simulink model "HapticPaddle"  (R2025a)
settings: Solver=FixedStepAuto  StartTime=0.0  StopTime=10  FixedStep=0.0001  RelTol=1e-3  EnableMultiTasking=on
values from neighbouring files (symbols this model uses):
  B_eq = B_p + R^2*B_m    (= 0.00017775)    [main.m]
  g = 9.81    [main.m]
  J_eq = (J_p + R^2*(J_rotor + J_m))    (= 0.000485304)    [main.m]
  l = 0.0251    [main.m]
  m_p = 0.048    [main.m]
  phi_target = 10.00    (= 10)    [main.m]
  R = r_p1 / r_m    (= 15)    [main.m]
  r_p2 = 0.081    [main.m]
  Tau_f_dry = 0.00156    [main.m]
libraries: simulink_extras x3
settings Model: Creator=jemetzge  LastModifiedBy=tk
settings SolverCC: AlgebraicLoopSolver=TrustRegion
settings DataIOCC: LimitDataPoints=on  SaveFormat=Array  SignalLoggingSaveFormat=ModelDataLogs  ReturnWorkspaceOutputs=off
settings OptimizationCC: ExpressionDepthLimit=2147483647.0  LifeSpan=inf
settings DebuggingCC: UnderspecifiedInitializationDetection=Classic  MergeDetectMultiDrivingBlocksExec=none  SolverPrmCheckMsg=warning  FcnCallInpInsideContextMsg=warning  UnconnectedInputMsg=warning  UnconnectedOutputMsg=warning  UnconnectedLineMsg=warning  StateNameClashWarn=warning  SFUnexpectedBacktrackingDiag=warning  SFNoUnconditionalDefaultTransitionDiag=warning  SFExecutionAtInitializationDiag=none  ArithmeticOperatorsInVariantConditions=warning
settings HardwareCC: ProdBitPerPointer=32.0  ProdBitPerSizeT=32.0  ProdBitPerPtrDiffT=32.0  ProdLargestAtomicFloat=None  ProdIntDivRoundTo=Undefined  ProdEndianess=Unspecified  ProdWordSize=32.0  ProdHWDeviceType=32-bit Generic
settings ModelReferenceCC: EnableRefExpFcnMdlSchedulingChecks=on  PropagateSignalLabelsOutOfModel=off
settings SFSimCC: SimUseLocalCustomCode=off  CustomCodeUndefinedFunction=UseInterfaceOnly
settings RTWCC: RTWUseLocalCustomCode=off  GPUComputeCapability=3.5
settings CodeAppCC: StateflowObjectComments=on
settings GRTTargetCC: TargetLangStandard=C89/C90 (ANSI)  CombineOutputUpdateFcns=off  GRTInterface=on
settings ConfigComp: CovMetricSettings=dw  CovSaveCumulativeToWorkspaceVar=on  CovSaveSingleToWorkspaceVar=on  CovExternalEMLEnable=off  CovSFcnEnable=off

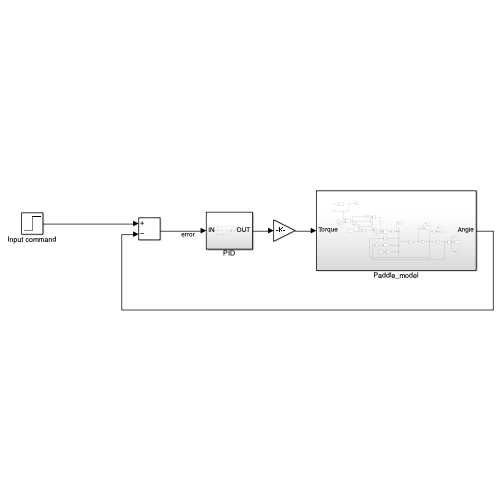
[thumbnail: Simulink's stored preview of the top-level diagram]
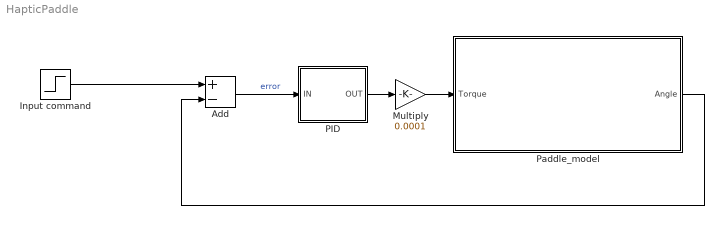
== system HapticPaddle ==
  Add : Sum  Inputs=+-
  Input command : Step  After=phi_target  SampleTime=0
  Multiply : Gain  Gain=0.0001
  PID : Subsystem
  Paddle_model : Subsystem
  wires:
  PID/1(OUT) -> Multiply/1
  Add/1 -> PID/1(IN)  "error"
  Paddle_model/1(Angle) -> Add/2
  Input command/1 -> Add/1
  Multiply/1 -> Paddle_model/1(Torque)

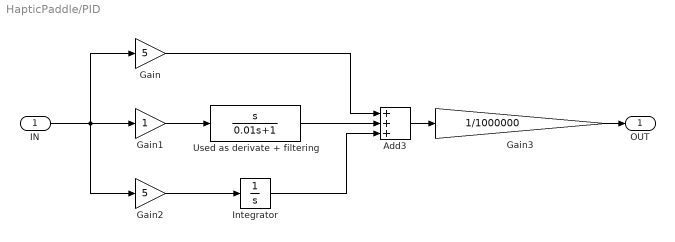
== system HapticPaddle/PID ==
  IN : Inport
  Add3 : Sum  Inputs=+++
  Gain : Gain  Gain=5
  Gain1 : Gain
  Gain2 : Gain  Gain=5
  Gain3 : Gain  Gain=1/1000000
  Integrator : Integrator
  Used as derivate + filtering : TransferFcn  Numerator=[1 0]  Denominator=[0.01 1]
  OUT : Outport
  wires:
  Integrator/1 -> Add3/3
  Gain2/1 -> Integrator/1
  Gain/1 -> Add3/1
  Gain3/1 -> OUT/1
  Gain1/1 -> Used as derivate + filtering/1
  Add3/1 -> Gain3/1
  Used as derivate + filtering/1 -> Add3/2
  IN/1 -> Gain2/1, Gain1/1, Gain/1

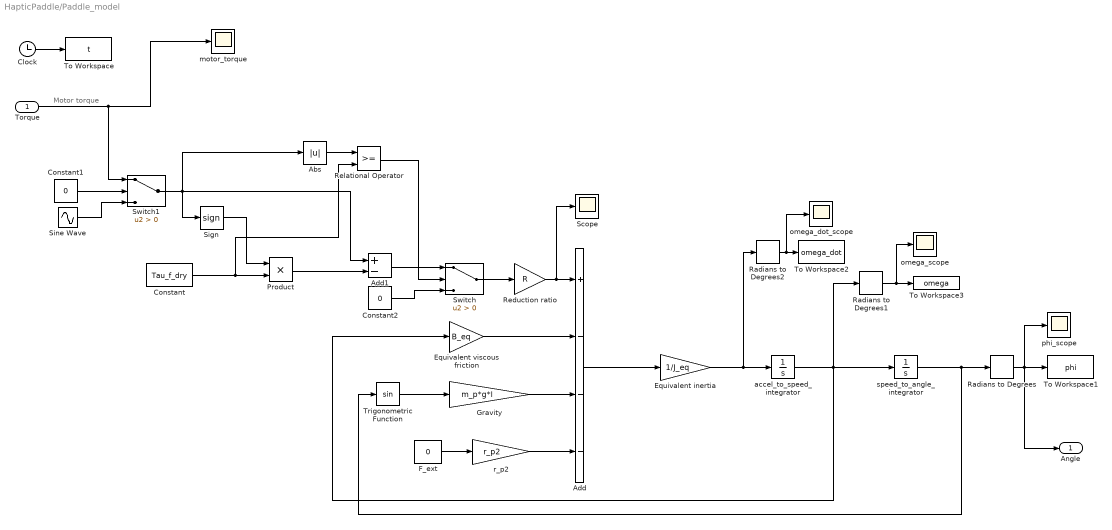
== system HapticPaddle/Paddle_model ==
  note: Motor torque
  Torque : Inport
  Abs : Abs  SaturateOnIntegerOverflow=off
  Add : Sum  Inputs=+---
  Add1 : Sum  Inputs=+-
  Clock : Clock
  Constant : Constant  Value=Tau_f_dry
  Constant1 : Constant  Value=0
  Constant2 : Constant  Value=0
  Equivalent inertia : Gain  Gain=1/J_eq
  Equivalent viscous friction : Gain  Gain=B_eq
  F_ext : Constant  Value=0
  Gravity : Gain  Gain=m_p*g*l
  Product : Product
  Radians to Degrees : simulink_extras/Transformations/Radians to Degrees
  Radians to Degrees1 : simulink_extras/Transformations/Radians to Degrees
  Radians to Degrees2 : simulink_extras/Transformations/Radians to Degrees
  Reduction ratio : Gain  Gain=R
  Relational Operator : RelationalOperator  OutDataTypeStr=boolean  RndMeth=Simplest  InputSameDT=off
  Scope : Scope
      settings: ActiveDisplayYMinimum=-1  ActiveDisplayYMaximum=1  DataLoggingVariableName=ScopeData4
  Sign : Signum
  Sine Wave : Sin  Amplitude=0.002  Frequency=2*pi*0.5  SampleTime=0
  Switch : Switch  Criteria=u2 > Threshold  SaturateOnIntegerOverflow=off  InputSameDT=off
  Switch1 : Switch  Criteria=u2 > Threshold  SaturateOnIntegerOverflow=off  InputSameDT=off
  To Workspace : ToWorkspace  VariableName=t  SampleTime=-1
  To Workspace1 : ToWorkspace  VariableName=phi  SampleTime=-1
  To Workspace2 : ToWorkspace  VariableName=omega_dot  SampleTime=-1
  To Workspace3 : ToWorkspace  VariableName=omega  SampleTime=-1
  Trigonometric Function : Trigonometry
  accel_to_speed_integrator : Integrator
  motor_torque : Scope
      settings: ActiveDisplayYMinimum=-1  ActiveDisplayYMaximum=1  DataLoggingVariableName=ScopeData3
  omega_dot_scope : Scope
      settings: ActiveDisplayYMinimum=-1  ActiveDisplayYMaximum=1  DataLoggingVariableName=ScopeData2
  omega_scope : Scope
      settings: ActiveDisplayYMinimum=-1  ActiveDisplayYMaximum=1
  phi_scope : Scope
  r_p2 : Gain  Gain=r_p2
  speed_to_angle_integrator : Integrator
  Angle : Outport
  wires:
  r_p2/1 -> Add/4
  Add/1 -> Equivalent inertia/1
  Clock/1 -> To Workspace/1
  Equivalent inertia/1 -> Radians to Degrees2/1, accel_to_speed_integrator/1
  Radians to Degrees/1 -> Angle/1, phi_scope/1, To Workspace1/1
  Gravity/1 -> Add/3
  F_ext/1 -> r_p2/1
  Torque/1 -> motor_torque/1, Switch1/1
  Radians to Degrees2/1 -> omega_dot_scope/1, To Workspace2/1
  accel_to_speed_integrator/1 -> Radians to Degrees1/1, Equivalent viscous friction/1, speed_to_angle_integrator/1
  Trigonometric Function/1 -> Gravity/1
  Radians to Degrees1/1 -> omega_scope/1, To Workspace3/1
  Equivalent viscous friction/1 -> Add/2
  speed_to_angle_integrator/1 -> Radians to Degrees/1, Trigonometric Function/1
  Reduction ratio/1 -> Scope/1, Add/1
  Add1/1 -> Switch/1
  Product/1 -> Add1/2
  Constant/1 -> Relational Operator/2, Product/2
  Sign/1 -> Product/1
  Switch/1 -> Reduction ratio/1
  Switch1/1 -> Sign/1, Add1/1, Abs/1
  Sine Wave/1 -> Switch1/3
  Constant1/1 -> Switch1/2
  Constant2/1 -> Switch/3
  Abs/1 -> Relational Operator/1
  Relational Operator/1 -> Switch/2
